simulink library "lib_AC_IG"  (R2026a)
settings: Solver=VariableStepAuto
undefined symbols (not defined in the file): block_buses, block_idx, block_toM, buses_lf, fref, invL, op_IG
settings Model: Creator=atomas  LastModifiedBy=atomas

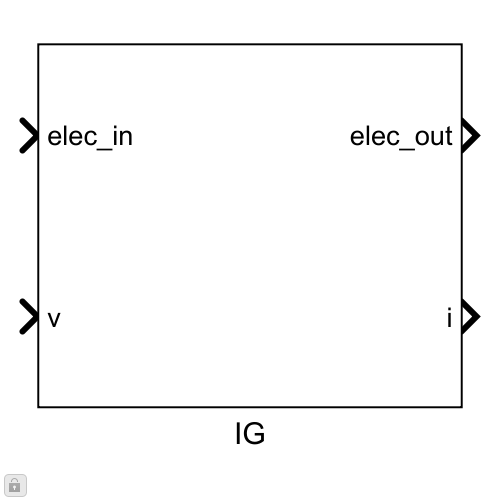
[thumbnail: Simulink's stored preview of the top-level diagram]
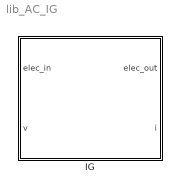
== system lib_AC_IG ==
  IG : Subsystem  mask{L_out_pu=0.1, R_out_pu=0.01}
      mask init:
      | [block_buses, block_idx, block_toM, block_fref] = mask_init_IG(gcb);

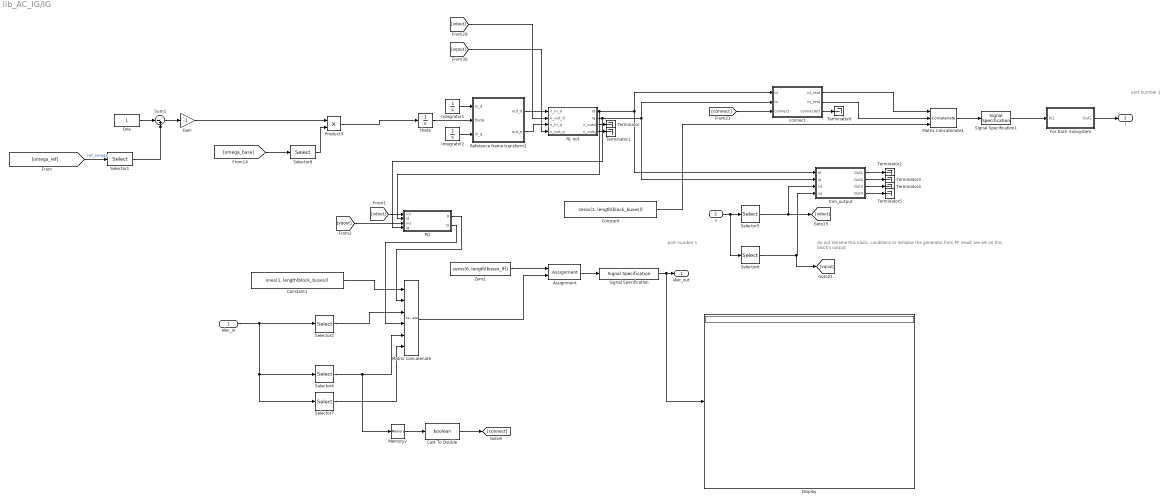
== system lib_AC_IG/IG ==
  note: do not rename this block, conditions to initialise the generator from PF result are set on this block's output
  note: port number 1
  note: port number 2
  elec_in : Inport
  v : Inport  Port=2
  Assignment : Assignment  NumberOfDimensions=2  DiagnosticForDimensions=Warning  IndexOptions=Assign all,Index vector (dialog)  Indices=1,block_idx  OutputSizes=1,1
  Cast To Double : DataTypeConversion  OutDataTypeStr=boolean  SaturateOnIntegerOverflow=off  RndMeth=Floor
  Constant : Constant  Value=zeros(1, length(block_buses))  VectorParams1D=off
  Constant1 : Constant  Value=ones(1, length(block_buses))  VectorParams1D=off
  Display : Display
  For Each Subsystem : Subsystem  TreatAsAtomicUnit=on
  Gain : Gain  Gain=-1
  Integrator1 : Integrator  InitialCondition=op_IG.Integrator1
  Integrator2 : Integrator  InitialCondition=op_IG.Integrator2
  Matrix Concatenate : Concatenate  NumInputs=6  Mode=Multidimensional array
  Matrix Concatenate1 : Concatenate  NumInputs=3  Mode=Multidimensional array
  Memory2 : Memory  InitialCondition=1
  One : Constant  OutDataTypeStr=Inherit: Inherit via back propagation
  PQ : Subsystem
  Product3 : Product
  RL out : Subsystem  Variant=on  mask{dynamic=Dynamic, R=1e-6, L=1e-6}
      mask prompts: dynamic "Dynamic behavior"; R "Series resistance (p.u.)"; L "Inductance (p.u.)"
      mask init:
      | [invL, omegab, rl_mode] = mask_init_RL(dynamic, L, 50);
      mask TypeOptions dynamic: Static | Dynamic | Static omega
  Reference frame transform2 : Subsystem
  Selector1 : Selector  InputPortWidth=length(fref.ref_units)  IndexOptions=Index vector (dialog)  Indices=block_fref  OutputSizes=1
  Selector2 : Selector  NumberOfDimensions=2  InputPortWidth=3  IndexOptions=Index vector (dialog),Index vector (dialog)  Indices=3,block_idx  OutputSizes=1,1
  Selector4 : Selector  NumberOfDimensions=2  InputPortWidth=3  IndexOptions=Index vector (dialog),Index vector (dialog)  Indices=5,block_idx  OutputSizes=1,1
  Selector5 : Selector  NumberOfDimensions=2  InputPortWidth=3  IndexOptions=Index vector (dialog),Index vector (dialog)  Indices=1,block_buses  OutputSizes=1,1
  Selector6 : Selector  NumberOfDimensions=2  InputPortWidth=3  IndexOptions=Index vector (dialog),Index vector (dialog)  Indices=2,block_buses  OutputSizes=1,1
  Selector7 : Selector  NumberOfDimensions=2  InputPortWidth=3  IndexOptions=Index vector (dialog),Index vector (dialog)  Indices=6,block_idx  OutputSizes=1,1
  Selector8 : Selector  InputPortWidth=length(fref.ref_units)  IndexOptions=Index vector (dialog)  Indices=block_fref  OutputSizes=1
  Signal Specification : SignalSpecification  Dimensions=[6 length(buses_lf)]
  Signal Specification1 : SignalSpecification  Dimensions=[3 length(block_buses)]
  Sum1 : Sum  Inputs=|-+
  Terminator{,1..6} (7 alike) : Terminator
  Zero1 : Constant  Value=zeros(6, length(buses_lf))  VectorParams1D=off  OutDataTypeStr=Inherit: Inherit via back propagation
  connect : Subsystem
  theta : Integrator  InitialCondition=op_IG.theta  UpperSaturationLimit=2*pi  LowerSaturationLimit=0
  trim_output : Subsystem
  elec_out : Outport
  i : Outport  Port=2
  wires:
  [vqout] -> RL out/4(v_out_q)
  RL out/3(v_outd) -> Terminator/1
  RL out/4(v_outq) -> Terminator1/1
  Reference frame transform2/1(out_d) -> RL out/1(v_in_d)
  Reference frame transform2/2(out_q) -> RL out/3(v_in_q)
  theta/1 -> Reference frame transform2/2(theta)
  Integrator1/1 -> Reference frame transform2/1(in_d)
  Integrator2/1 -> Reference frame transform2/3(in_q)
  Product3/1 -> theta/1
  Sum1/1 -> Gain/1
  [omega_ref] -> Selector1/1  "ref_omega"
  One/1 -> Sum1/1
  [vdout] -> RL out/2(v_out_d)
  RL out/1(id) -> PQ/2(id), connect/1(id), trim_output/1(id)
  RL out/2(iq) -> PQ/4(iq), connect/2(iq), trim_output/2(iq)
  Matrix Concatenate1/1 -> Signal Specification1/1
  Signal Specification1/1 -> For Each Subsystem/1(In1)
  Constant/1 -> Matrix Concatenate1/3
  For Each Subsystem/1(Out1) -> i/1
  trim_output/3(Out3) -> Terminator4/1
  trim_output/1(Out1) -> Terminator2/1
  trim_output/4(Out4) -> Terminator5/1
  trim_output/2(Out2) -> Terminator3/1
  v/1 -> Selector6/1, Selector5/1
  Selector5/1 -> [vdout], trim_output/3(vd)
  Selector6/1 -> [vqout], trim_output/4(vq)
  elec_in/1 -> Selector7/1, Selector4/1, Selector2/1
  Matrix Concatenate/1 -> Assignment/2
  Zero1/1 -> Assignment/1
  Assignment/1 -> Signal Specification/1
  Constant1/1 -> Matrix Concatenate/1
  Selector2/1 -> Matrix Concatenate/3
  Selector4/1 -> Memory2/1, Matrix Concatenate/5
  Selector7/1 -> Matrix Concatenate/6
  Signal Specification/1 -> Display/1, elec_out/1
  [vdout] -> PQ/1(vd)
  [vqout] -> PQ/3(vq)
  PQ/1(P) -> Matrix Concatenate/2
  PQ/2(Q) -> Matrix Concatenate/4
  [omega_base] -> Selector8/1
  Selector8/1 -> Product3/2
  Selector1/1 -> Sum1/2
  Memory2/1 -> Cast To Double/1
  [connect] -> connect/3(connect)
  connect/2(iq_real) -> Matrix Concatenate1/2
  connect/1(id_real) -> Matrix Concatenate1/1
  connect/3(connected) -> Terminator6/1
  Cast To Double/1 -> [connect]
  Gain/1 -> Product3/1

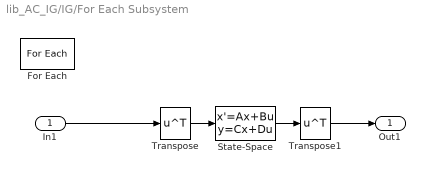
== system lib_AC_IG/IG/For Each Subsystem ==
  In1 : Inport  Partition=on  PartitionDimension=1  PartitionWidth=1  PartitionOffset=0
  For Each : ForEach  DisableCoverage=on
  State-Space : StateSpace  A=[]  B=[]  C=[]  D=block_toM  InitialCondition=0  ParameterTunability=Optimized
  Transpose : Math  Operator=transpose
  Transpose1 : Math  Operator=transpose
  Out1 : Outport  ConcatenationDimension=1
  wires:
  Transpose1/1 -> Out1/1
  In1/1 -> Transpose/1
  Transpose/1 -> State-Space/1
  State-Space/1 -> Transpose1/1

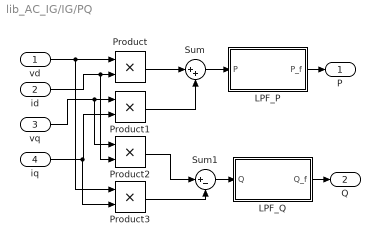
== system lib_AC_IG/IG/PQ ==
  vd : Inport
  id : Inport  Port=2
  vq : Inport  Port=3
  iq : Inport  Port=4
  LPF_P : Subsystem
  LPF_Q : Subsystem
  Product{,1..3} (4 alike) : Product
  Sum : Sum  Inputs=|++
  Sum1 : Sum  Inputs=|+-
  P : Outport
  Q : Outport  Port=2
  wires:
  Product/1 -> Sum/1
  Sum/1 -> LPF_P/1(P)
  vd/1 -> Product3/1, Product/1
  id/1 -> Product2/2, Product/2
  vq/1 -> Product2/1, Product1/1
  iq/1 -> Product3/2, Product1/2
  Product1/1 -> Sum/2
  Sum1/1 -> LPF_Q/1(Q)
  Product2/1 -> Sum1/1
  Product3/1 -> Sum1/2
  LPF_P/1(P_f) -> P/1
  LPF_Q/1(Q_f) -> Q/1

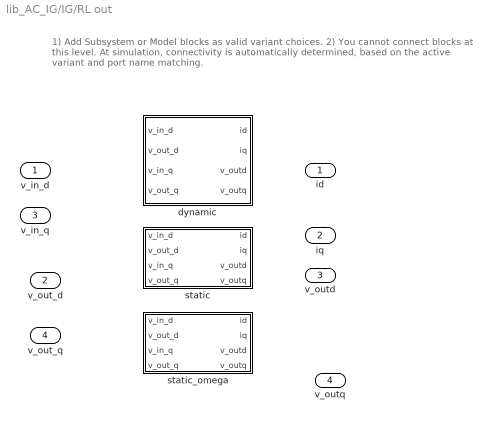
== system lib_AC_IG/IG/RL out ==
  note: 1) Add Subsystem or Model blocks as valid variant choices.
      | 2) You cannot connect blocks at this level. At simulation, connectivity is automatically
      | determined, based on the active variant and port name matching.
  v_in_d : Inport
  v_out_d : Inport  Port=2
  v_in_q : Inport  Port=3
  v_out_q : Inport  Port=4
  dynamic : Subsystem  VariantControl=rl_mode == 1
  static : Subsystem  VariantControl=rl_mode == 2
  static_omega : Subsystem  VariantControl=(default)
  id : Outport
  iq : Outport  Port=2
  v_outd : Outport  Port=3
  v_outq : Outport  Port=4

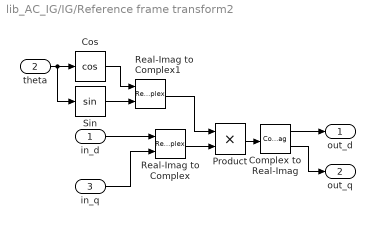
== system lib_AC_IG/IG/Reference frame transform2 ==
  in_d : Inport
  theta : Inport  Port=2
  in_q : Inport  Port=3
  Complex to Real-Imag : ComplexToRealImag
  Cos : Trigonometry  SCDEnableBlockLinearizationSpecification=on  Operator=cos
  Product : Product
  Real-Imag to Complex : RealImagToComplex
  Real-Imag to Complex1 : RealImagToComplex
  Sin : Trigonometry  SCDEnableBlockLinearizationSpecification=on
  out_d : Outport
  out_q : Outport  Port=2
  wires:
  in_d/1 -> Real-Imag to Complex/1
  in_q/1 -> Real-Imag to Complex/2
  Complex to Real-Imag/1 -> out_d/1
  Sin/1 -> Real-Imag to Complex1/2
  Cos/1 -> Real-Imag to Complex1/1
  theta/1 -> Cos/1, Sin/1
  Product/1 -> Complex to Real-Imag/1
  Real-Imag to Complex/1 -> Product/2
  Real-Imag to Complex1/1 -> Product/1
  Complex to Real-Imag/2 -> out_q/1

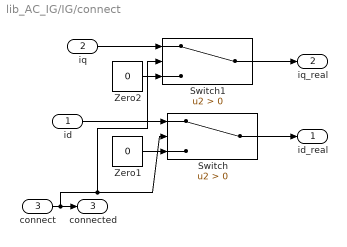
== system lib_AC_IG/IG/connect ==
  id : Inport
  iq : Inport  Port=2
  connect : Inport  Port=3
  Switch : Switch  Criteria=u2 > Threshold  ZeroCross=off  SaturateOnIntegerOverflow=off  InputSameDT=off
  Switch1 : Switch  Criteria=u2 > Threshold  ZeroCross=off  SaturateOnIntegerOverflow=off  InputSameDT=off
  Zero1 : Constant  Value=0  VectorParams1D=off  OutDataTypeStr=Inherit: Inherit via back propagation
  Zero2 : Constant  Value=0  VectorParams1D=off  OutDataTypeStr=Inherit: Inherit via back propagation
  id_real : Outport
  iq_real : Outport  Port=2
  connected : Outport  Port=3  OutDataTypeStr=boolean
  wires:
  Switch/1 -> id_real/1
  Zero1/1 -> Switch/3
  id/1 -> Switch/1
  connect/1 -> connected/1, Switch1/2, Switch/2
  Switch1/1 -> iq_real/1
  iq/1 -> Switch1/1
  Zero2/1 -> Switch1/3

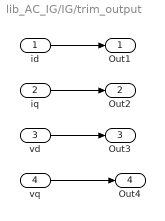
== system lib_AC_IG/IG/trim_output ==
  id : Inport
  iq : Inport  Port=2
  vd : Inport  Port=3
  vq : Inport  Port=4
  Out1 : Outport
  Out2 : Outport  Port=2
  Out3 : Outport  Port=3
  Out4 : Outport  Port=4
  wires:
  id/1 -> Out1/1
  vq/1 -> Out4/1
  vd/1 -> Out3/1
  iq/1 -> Out2/1

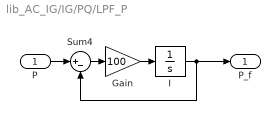
== system lib_AC_IG/IG/PQ/LPF_P ==
  P : Inport
  Gain : Gain  Gain=100
  I : Integrator  InitialCondition=op_IG.PQ_LPF_P_I
  Sum4 : Sum  Inputs=|+-
  P_f : Outport
  wires:
  Gain/1 -> I/1
  Sum4/1 -> Gain/1
  P/1 -> Sum4/1
  I/1 -> P_f/1, Sum4/2

== system lib_AC_IG/IG/PQ/LPF_Q ==
  Q : Inport
  Gain : Gain  Gain=100
  I : Integrator  InitialCondition=op_IG.PQ_LPF_Q_I
  Sum4 : Sum  Inputs=|+-
  Q_f : Outport
  wires:
  Gain/1 -> I/1
  Q/1 -> Sum4/1
  I/1 -> Q_f/1, Sum4/2
  Sum4/1 -> Gain/1

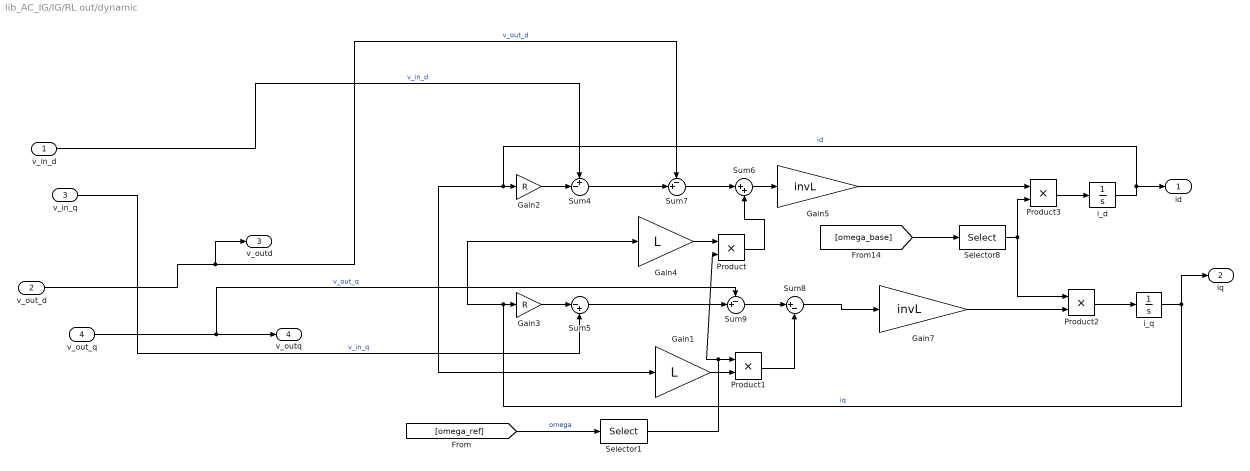
== system lib_AC_IG/IG/RL out/dynamic ==
  v_in_d : Inport
  v_out_d : Inport  Port=2
  v_in_q : Inport  Port=3
  v_out_q : Inport  Port=4
  Gain1 : Gain  Gain=L
  Gain2 : Gain  Gain=R
  Gain3 : Gain  Gain=R
  Gain4 : Gain  Gain=L
  Gain5 : Gain  Gain=invL
  Gain7 : Gain  Gain=invL
  Product{,1..3} (4 alike) : Product
  Selector1 : Selector  InputPortWidth=length(fref.ref_units)  IndexOptions=Index vector (dialog)  Indices=block_fref  OutputSizes=1
  Selector8 : Selector  InputPortWidth=length(fref.ref_units)  IndexOptions=Index vector (dialog)  Indices=block_fref  OutputSizes=1
  Sum4 : Sum  Inputs=+-|
  Sum5 : Sum  Inputs=|-+
  Sum6 : Sum  Inputs=|++
  Sum7 : Sum  Inputs=-+|
  Sum8 : Sum  Inputs=|+-
  Sum9 : Sum  Inputs=-+|
  i_d : Integrator  InitialCondition=op_IG.RL_out_dynamic_i_d
  i_q : Integrator  InitialCondition=op_IG.RL_out_dynamic_i_q
  id : Outport
  iq : Outport  Port=2
  v_outd : Outport  Port=3
  v_outq : Outport  Port=4
  wires:
  v_out_q/1 -> v_outq/1, Sum9/1  "v_out_q"
  v_out_d/1 -> v_outd/1, Sum7/1  "v_out_d"
  Sum9/1 -> Sum8/1
  Gain1/1 -> Product1/2
  i_q/1 -> iq/1, Gain4/1, Gain3/1  "iq"
  Sum5/1 -> Sum9/2
  Gain3/1 -> Sum5/1
  Sum7/1 -> Sum6/1
  Gain4/1 -> Product/1
  Product1/1 -> Sum8/2
  Sum4/1 -> Sum7/2
  Sum8/1 -> Gain7/1
  Product/1 -> Sum6/2
  [omega_ref] -> Selector1/1  "omega"
  Sum6/1 -> Gain5/1
  i_d/1 -> id/1, Gain1/1, Gain2/1  "id"
  Gain2/1 -> Sum4/2
  v_in_d/1 -> Sum4/1  "v_in_d"
  v_in_q/1 -> Sum5/2  "v_in_q"
  [omega_base] -> Selector8/1
  Selector8/1 -> Product2/1, Product3/2
  Product3/1 -> i_d/1
  Product2/1 -> i_q/1
  Gain7/1 -> Product2/2
  Selector1/1 -> Product/2, Product1/1
  Gain5/1 -> Product3/1

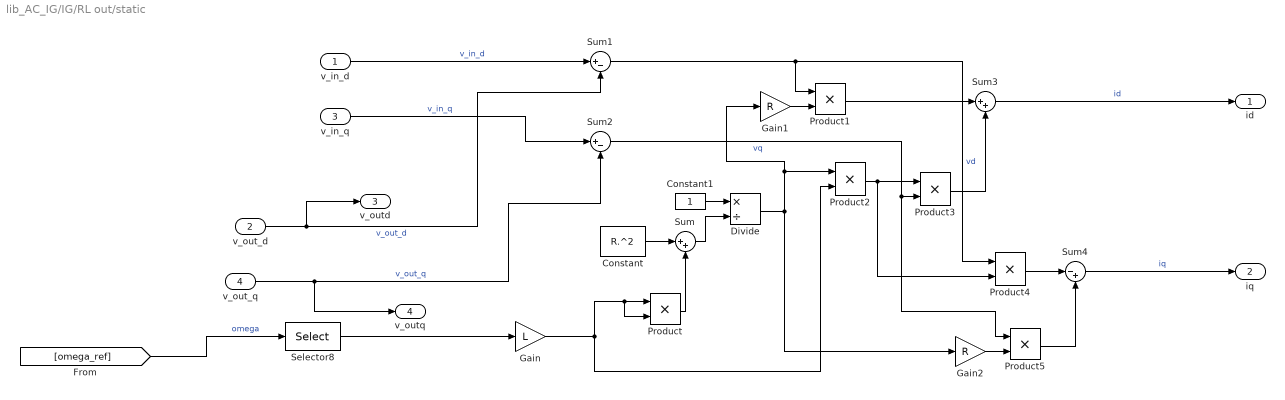
== system lib_AC_IG/IG/RL out/static ==
  v_in_d : Inport
  v_out_d : Inport  Port=2
  v_in_q : Inport  Port=3
  v_out_q : Inport  Port=4
  Constant : Constant  Value=R.^2
  Constant1 : Constant
  Divide : Product  Inputs=*/
  Gain : Gain  Gain=L
  Gain1 : Gain  Gain=R
  Gain2 : Gain  Gain=R
  Product{,1..5} (6 alike) : Product
  Selector8 : Selector  InputPortWidth=length(fref.ref_units)  IndexOptions=Index vector (dialog)  Indices=block_fref  OutputSizes=1
  Sum : Sum  Inputs=|++
  Sum1 : Sum  Inputs=|+-
  Sum2 : Sum  Inputs=|+-
  Sum3 : Sum  Inputs=|++
  Sum4 : Sum  Inputs=|-+
  id : Outport
  iq : Outport  Port=2
  v_outd : Outport  Port=3
  v_outq : Outport  Port=4
  wires:
  [omega_ref] -> Selector8/1  "omega"
  v_in_d/1 -> Sum1/1  "v_in_d"
  v_out_q/1 -> v_outq/1, Sum2/2  "v_out_q"
  Sum4/1 -> iq/1  "iq"
  Sum3/1 -> id/1  "id"
  Gain1/1 -> Product1/2
  Product2/1 -> Product4/2, Product3/1
  Product4/1 -> Sum4/1
  Divide/1 -> Gain2/1, Gain1/1, Product2/1
  Sum1/1 -> Product1/1, Product4/1  "vd"
  Product3/1 -> Sum3/2
  Constant1/1 -> Divide/1
  Gain/1 -> Product/2, Product/1, Product2/2
  Sum2/1 -> Product5/1, Product3/2  "vq"
  Constant/1 -> Sum/1
  Product5/1 -> Sum4/2
  Product1/1 -> Sum3/1
  Product/1 -> Sum/2
  Gain2/1 -> Product5/2
  Sum/1 -> Divide/2
  v_out_d/1 -> v_outd/1, Sum1/2  "v_out_d"
  v_in_q/1 -> Sum2/1  "v_in_q"
  Selector8/1 -> Gain/1

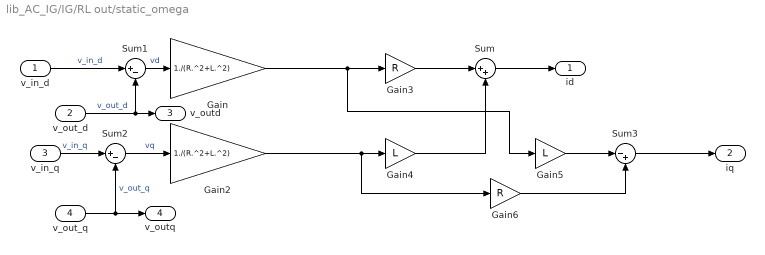
== system lib_AC_IG/IG/RL out/static_omega ==
  v_in_d : Inport
  v_out_d : Inport  Port=2
  v_in_q : Inport  Port=3
  v_out_q : Inport  Port=4
  Gain : Gain  Gain=1./(R.^2+L.^2)
  Gain2 : Gain  Gain=1./(R.^2+L.^2)
  Gain3 : Gain  Gain=R
  Gain4 : Gain  Gain=L
  Gain5 : Gain  Gain=L
  Gain6 : Gain  Gain=R
  Sum : Sum  Inputs=|++
  Sum1 : Sum  Inputs=|+-
  Sum2 : Sum  Inputs=|+-
  Sum3 : Sum  Inputs=|-+
  id : Outport
  iq : Outport  Port=2
  v_outd : Outport  Port=3
  v_outq : Outport  Port=4
  wires:
  v_in_q/1 -> Sum2/1  "v_in_q"
  v_in_d/1 -> Sum1/1  "v_in_d"
  v_out_q/1 -> v_outq/1, Sum2/2  "v_out_q"
  v_out_d/1 -> v_outd/1, Sum1/2  "v_out_d"
  Sum1/1 -> Gain/1  "vd"
  Sum2/1 -> Gain2/1  "vq"
  Gain/1 -> Gain5/1, Gain3/1
  Gain3/1 -> Sum/1
  Gain4/1 -> Sum/2
  Gain2/1 -> Gain6/1, Gain4/1
  Sum/1 -> id/1
  Gain5/1 -> Sum3/1
  Sum3/1 -> iq/1
  Gain6/1 -> Sum3/2
